simulink model "BEV"  (R2019b)
settings: Solver=ode4  StartTime=0.0  StopTime=TimeUS06  FixedStep=.1  RelTol=1e-3  EnableMultiTasking=on
PostLoadFcn:
  | addpath('ImagesBEV')
  | 
  | BEVDir = pwd;
  | 
  | cd ..\;
  | SimulinkDir = pwd;
  | addpath(SimulinkDir);
  | 
  | cd(BEVDir);
StopFcn:
  | MotorNetTorque = results.Motor.MotorNetTorque_Nm_;
  | SOC = results.Battery.SOC___;
  | BatteryPowerAtTerminals = results.Battery.BatteryPowerAtTerminals_W_;
  | VehicleSpeed = results.Glider.Velocity_mph_;
  | 
  | figure
  | scatter(VehicleSpeed.get.Data(:),MotorNetTorque.get.Data(:),'.')
  | grid on
  | box on
  | title('Motor Torque vs. Vehicle Speed')
  | xlabel('Vehicle Speed, V (mph)')
  | ylabel('Motor Torque, Tm (Nm)')
  | 
  | figure
  | scatter(VehicleSpeed.get.Data(:),BatteryPowerAtTerminals.get.Data(:))
  | grid on
  | box on
  | title('Battery Power vs. Vehicle Speed')
  | xlabel('Vehicle Speed, (mph)')
  | ylabel('Power, (kW)')
  | 
  | figure
  | plot(SOC.get.Time(:),SOC.get.Data(:))
  | grid on
  | box on
  | title('SOC vs. Time')
  | xlabel('Time (s)')
  | ylabel('SOC (%)')
  | 
  | clear MotorNetTorque SOC BatteryPowerAtTerminals VehicleSpeed ;
model workspace (MAT data in the model file):
  AccessoryLoad = 600
  C_ref = 600
  DrCycles.C505 = [0 1 2 3 4 5 6 7 8 9 10 11 ... (1012 elements, 506x2)]
  DrCycles.FTP = [0 1 2 3 4 5 6 7 8 9 10 11 ... (4956 elements, 2478x2)]
  DrCycles.UDDS = [0 1 2 3 4 5 6 7 8 9 10 11 ... (2746 elements, 1373x2)]
  DrCycles.HWFET = [0 1 2 3 4 5 6 7 8 9 10 11 ... (1532 elements, 766x2)]
  DrCycles.US06 = [0 1 2 3 4 5 6 7 8 9 10 11 ... (1194 elements, 597x2)]
  DrCycles.US06City = [0 1 2 3 4 5 6 7 8 9 10 11 ... (466 elements, 233x2)]
  DrCycles.US06Hwy = [0 1 2 3 4 5 6 7 8 9 10 11 ... (742 elements, 371x2)]
  K = 1.04716227018
  Kc_ref = 0.12
  Ki_ref = 0.01
  Kw_ref = 1.2e-05
  MDL.MotorModel.kc = 0.0452374100719
  MDL.MotorModel.ki = 0.0166666666667
  MDL.MotorModel.kw = 5.06640055941e-05
  MDL.MotorModel.C = 628.29736211
  MDL.MotorModel.MaxTrqOut = 500
  MDL.MotorModel.MaxPwrOut = 100000
  MDL.DrivelineModel.C0 = 600
  MDL.DrivelineModel.C1 = 0.012
  MDL.DrivelineModel.C2 = 4.9e-07
  MDL.DrivelineModel.G = 3.55
  MDL.DrivelineModel.Spinloss = 6
  MDL.DrivelineModel.Ftr_max = 5000
  MDL.DriverModel.Kp = 350
  MDL.DriverModel.Ki = 0
  MDL.DriverModel.Kd = 0
  MDL.DriverModel.BrakeGain = 100
  MDL.DriverModel.Ftr_Max = 5000
  MDL.DriverModel.Ptr_Max = 100000
  MDL.BrakeSys.MaxBrakeForce = 10000
  MDL.BrakeSys.RegenFraction = 0.55
  T_max = 500
  T_ref = 300
  TimeHWFET = 765
  TimeUDDS = 1372
  TimeUS06 = 596
  aeroDragCoeff = 0.38
  airDensity = 1.23
  energyCapacity = 12.6
  frontArea = 2.1
  gravity = 9.81
  inclinationAngle = 0
  inertialMassVeh = 2392
  initialSOC = 0.95
  internalResistance = 0.1
  massVeh = 2300
  openCircuitVoltage = 340
  rollingResistCoeff = 0.01
  w_max = 524
  w_ref = 834
  wheelRadius = 0.34
libraries: simulink x5, Driver_Glider_Library x2
CloseFcn:
  | rmpath(SimulinkDir);
  | rmpath('ImagesBEV')
  | clear BEVDir SimulinkDir;
settings Model: Creator=David  LastModifiedBy=valakshe
settings DataIOCC: ExternalInput=DrCycles.US06  LoadExternalInput=on  SaveFormat=Array  ReturnWorkspaceOutputs=off
settings OptimizationCC: ExpressionDepthLimit=2147483647  LifeSpan=inf
settings DebuggingCC: UnderspecifiedInitializationDetection=Classic  MergeDetectMultiDrivingBlocksExec=none  SolverPrmCheckMsg=warning  FcnCallInpInsideContextMsg=warning  StateNameClashWarn=warning  SFUnexpectedBacktrackingDiag=warning  SFNoUnconditionalDefaultTransitionDiag=warning  SFExecutionAtInitializationDiag=none  ArithmeticOperatorsInVariantConditions=warning
settings HardwareCC: ProdBitPerPointer=32  ProdBitPerSizeT=32  ProdBitPerPtrDiffT=32  ProdLargestAtomicFloat=None  ProdIntDivRoundTo=Undefined  ProdEndianess=Unspecified  ProdWordSize=32  ProdHWDeviceType=32-bit Generic
settings ModelReferenceCC: PropagateSignalLabelsOutOfModel=off
settings SFSimCC: SimUseLocalCustomCode=off  CustomCodeUndefinedFunction=UseInterfaceOnly
settings RTWCC: RTWUseLocalCustomCode=off
settings CodeAppCC: StateflowObjectComments=on
settings GRTTargetCC: TargetLangStandard=C89/C90 (ANSI)  GeneratePreprocessorConditionals=Disable all  CombineOutputUpdateFcns=off  GRTInterface=on
settings ConfigComp: CovMetricSettings=dw  CovHtmlReporting=on  CovSaveCumulativeToWorkspaceVar=on  CovSaveSingleToWorkspaceVar=on  CovExternalEMLEnable=off  CovSFcnEnable=off

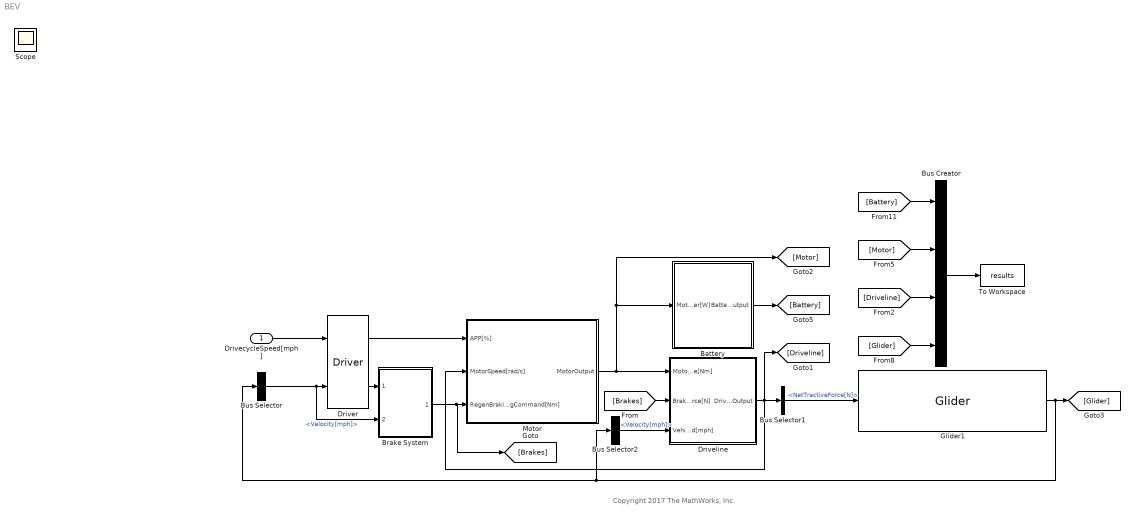
== system BEV ==
  note: Copyright 2017 The MathWorks, Inc.
  DrivecycleSpeed[mph] : Inport
  Battery : Subsystem
      mask Display: image('battery.jpg');
  Brake System : Subsystem
      mask Display: image('brakes.jpg');
  Bus Creator : BusCreator  Inputs=4
  Bus Selector : BusSelector  OutputSignals=Velocity[mph]
  Bus Selector1 : BusSelector  OutputSignals=NetTractiveForce[N]
  Bus Selector2 : BusSelector  OutputSignals=Velocity[mph]
  Driveline : Subsystem
      mask Display: image('driveline.jpg');
  Driver : Driver_Glider_Library/Driver  SystemSampleTime=-1  Latency=0  AutoFrameSizeCalculation=off
  Glider1 : Driver_Glider_Library/Glider  SystemSampleTime=-1  Latency=0  AutoFrameSizeCalculation=off
  Motor : Subsystem
      mask Display: image('motor.jpg');
  To Workspace : ToWorkspace  VariableName=results  SaveFormat=Timeseries  SampleTime=-1
  Scope : Scope
  wires:
  DrivecycleSpeed[mph]/1 -> Driver/1
  Driver/1 -> Motor/1(APP[%])
  Bus Creator/1 -> To Workspace/1
  Driver/2 -> Brake System/1(BPP[%])
  [Brakes] -> Driveline/2(BrakeForce[N])
  Brake System/1(BrakeOutput) -> [Brakes], Motor/3(RegenBrakingCommand[Nm])
  [Driveline] -> Bus Creator/3
  Driveline/1(DrivelineOutput) -> Bus Selector1/1, Motor/2(MotorSpeed[rad/s]), [Driveline]
  [Motor] -> Bus Creator/2
  Motor/1(MotorOutput) -> [Motor], Battery/1(MotorPower[W]), Driveline/1(MotorTorque[Nm])
  [Glider] -> Bus Creator/4
  Glider1/1 -> [Glider], Bus Selector/1, Bus Selector2/1
  Bus Selector/1 -> Brake System/2(VehicleSpeed[mph]), Driver/2  "<Velocity[mph]>"
  Bus Selector2/1 -> Driveline/3(VehicleSpeed[mph])  "<Velocity[mph]>"
  [Battery] -> Bus Creator/1
  Battery/1(BatteryOutput) -> [Battery]
  Bus Selector1/1 -> Glider1/1  "<NetTractiveForce[N]>"

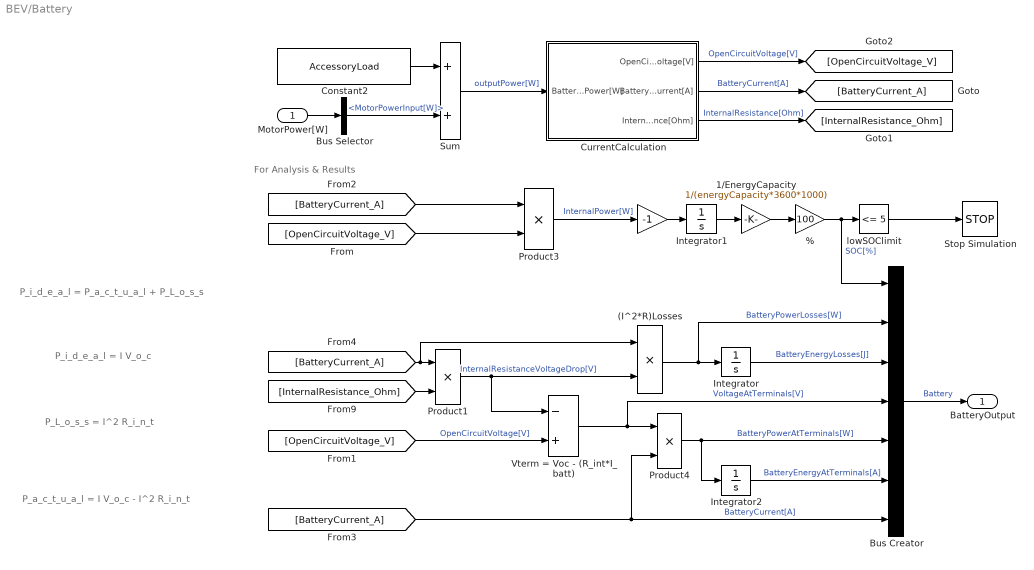
== system BEV/Battery ==
  note: For Analysis & Results
  note: P_i_d_e_a_l = I V_o_c
  note: P_i_d_e_a_l = P_a_c_t_u_a_l + P_L_o_s_s
  note: P_L_o_s_s = I^2 R_i_n_t
  note: P_a_c_t_u_a_l = I V_o_c - I^2 R_i_n_t
  MotorPower[W] : Inport
  " " : Gain  Gain=-1
  % : Gain  Gain=100
  (I^2*R)Losses : Product  RndMeth=Zero
  1/EnergyCapacity : Gain  Gain=1/(energyCapacity*3600*1000)
  Bus Creator : BusCreator  Inputs=7
  Bus Selector : BusSelector  OutputSignals=MotorPowerInput[W]
  Constant2 : Constant  Value=AccessoryLoad
  CurrentCalculation : Subsystem
  Integrator : Integrator  ZeroCross=off
  Integrator1 : Integrator  InitialCondition=energyCapacity*3600*1000*initialSOC  ZeroCross=off
  Integrator2 : Integrator
  Product1 : Product  RndMeth=Zero
  Product3 : Product  RndMeth=Zero
  Product4 : Product  RndMeth=Zero
  Stop Simulation : Stop
  Sum : Sum
  Vterm = Voc - (R_int*I_batt) : Sum  Inputs=-+
  lowSOClimit : simulink/Logic and Bit Operations/Compare To Constant  relop=<=  const=5  OutDataTypeStr=boolean
  BatteryOutput : Outport  VectorParamsAs1DForOutWhenUnconnected=off
  wires:
  Product1/1 -> (I^2*R)Losses/2, Vterm = Voc - (R_int*I_batt)/1  "InternalResistanceVoltageDrop[V]"
  (I^2*R)Losses/1 -> Bus Creator/2, Integrator/1  "BatteryPowerLosses[W]"
  Integrator/1 -> Bus Creator/3  "BatteryEnergyLosses[J]"
  Product3/1 -> " "/1  "InternalPower[W]"
  Integrator1/1 -> 1/EnergyCapacity/1
  Constant2/1 -> Sum/1
  Bus Creator/1 -> BatteryOutput/1  "Battery"
  1/EnergyCapacity/1 -> %/1
  MotorPower[W]/1 -> Bus Selector/1
  Sum/1 -> CurrentCalculation/1(BatteryPower[W])  "outputPower[W]"
  " "/1 -> Integrator1/1
  Bus Selector/1 -> Sum/2  "<MotorPowerInput[W]>"
  [OpenCircuitVoltage_V] -> Product3/2
  CurrentCalculation/1(OpenCircuitVoltage[V]) -> [OpenCircuitVoltage_V]  "OpenCircuitVoltage[V]"
  [OpenCircuitVoltage_V] -> Vterm = Voc - (R_int*I_batt)/2  "OpenCircuitVoltage[V]"
  [BatteryCurrent_A] -> Product3/1
  [BatteryCurrent_A] -> Bus Creator/7, Product4/2  "BatteryCurrent[A]"
  [BatteryCurrent_A] -> (I^2*R)Losses/1, Product1/1
  Vterm = Voc - (R_int*I_batt)/1 -> Bus Creator/4, Product4/1  "VoltageAtTerminals[V]"
  CurrentCalculation/2(BatteryCurrent[A]) -> [BatteryCurrent_A]  "BatteryCurrent[A]"
  CurrentCalculation/3(InternalResistance[Ohm]) -> [InternalResistance_Ohm]  "InternalResistance[Ohm]"
  [InternalResistance_Ohm] -> Product1/2
  Product4/1 -> Bus Creator/5, Integrator2/1  "BatteryPowerAtTerminals[W]"
  Integrator2/1 -> Bus Creator/6  "BatteryEnergyAtTerminals[A]"
  %/1 -> lowSOClimit/1, Bus Creator/1  "SOC[%]"
  lowSOClimit/1 -> Stop Simulation/1

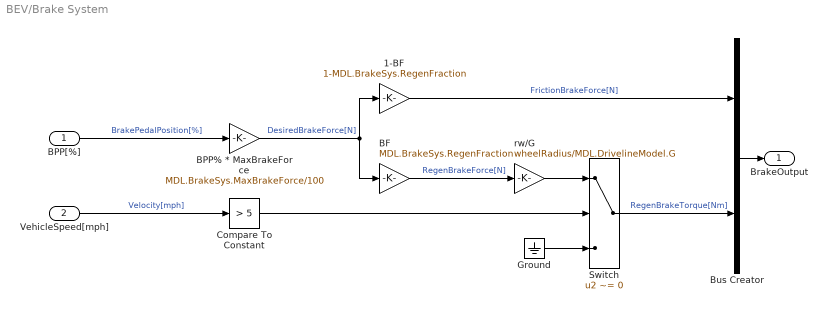
== system BEV/Brake System ==
  BPP[%] : Inport
  VehicleSpeed[mph] : Inport  Port=2
  1-BF : Gain  Gain=1-MDL.BrakeSys.RegenFraction
  BF : Gain  Gain=MDL.BrakeSys.RegenFraction
  BPP% * MaxBrakeForce : Gain  Gain=MDL.BrakeSys.MaxBrakeForce/100
  Bus Creator : BusCreator  Inputs=2
  Compare To Constant : simulink/Logic and Bit Operations/Compare To Constant  relop=>  const=5  OutDataTypeStr=boolean
  Ground : Ground
  Switch : Switch  Criteria=u2 ~= 0
  rw/G : Gain  Gain=wheelRadius/MDL.DrivelineModel.G
  BrakeOutput : Outport  VectorParamsAs1DForOutWhenUnconnected=off
  wires:
  Bus Creator/1 -> BrakeOutput/1
  BPP[%]/1 -> BPP% * MaxBrakeForce/1  "BrakePedalPosition[%]"
  BPP% * MaxBrakeForce/1 -> BF/1, 1-BF/1  "DesiredBrakeForce[N]"
  BF/1 -> rw/G/1  "RegenBrakeForce[N]"
  1-BF/1 -> Bus Creator/1  "FrictionBrakeForce[N]"
  rw/G/1 -> Switch/1
  VehicleSpeed[mph]/1 -> Compare To Constant/1  "Velocity[mph]"
  Ground/1 -> Switch/3
  Switch/1 -> Bus Creator/2  "RegenBrakeTorque[Nm]"
  Compare To Constant/1 -> Switch/2

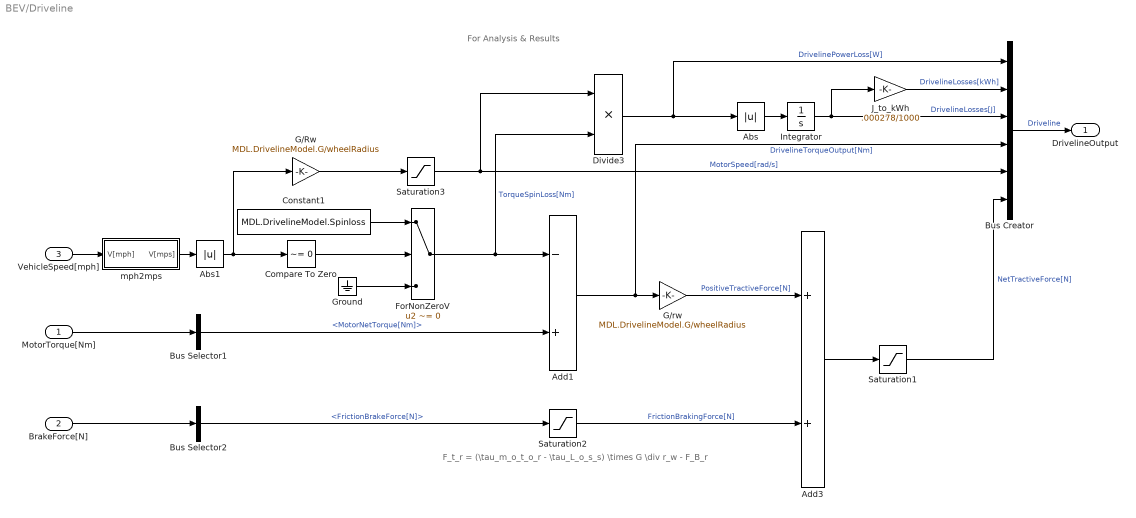
== system BEV/Driveline ==
  note: For Analysis & Results
  note: F_t_r = (\tau_m_o_t_o_r - \tau_L_o_s_s) \times G \div r_w - F_B_r
  MotorTorque[Nm] : Inport
  BrakeForce[N] : Inport  Port=2
  VehicleSpeed[mph] : Inport  Port=3
  Abs : Abs  ZeroCross=off
  Abs1 : Abs  ZeroCross=off
  Add1 : Sum  Inputs=-+
  Add3 : Sum
  Bus Creator : BusCreator  Inputs=6
  Bus Selector1 : BusSelector  OutputSignals=MotorNetTorque[Nm]
  Bus Selector2 : BusSelector  OutputSignals=FrictionBrakeForce[N]
  Compare To Zero : simulink/Logic and Bit Operations/Compare To Zero  relop=~=  OutDataTypeStr=boolean
  Constant1 : Constant  Value=MDL.DrivelineModel.Spinloss
  Divide3 : Product  Inputs=**
  ForNonZeroV : Switch  Criteria=u2 ~= 0  ZeroCross=off
  G/Rw : Gain  Gain=MDL.DrivelineModel.G/wheelRadius
  G/rw : Gain  Gain=MDL.DrivelineModel.G/wheelRadius
  Ground : Ground
  Integrator : Integrator  ZeroCross=off
  J_to_kWh : Gain  Gain=.000278/1000
  Saturation1 : Saturate  UpperLimit=5000  LowerLimit=-10000  ZeroCross=off
  Saturation2 : Saturate  UpperLimit=0  LowerLimit=-10000  ZeroCross=off
  Saturation3 : Saturate  UpperLimit=inf  LowerLimit=0.00001  ZeroCross=off
  mph2mps : Subsystem
  DrivelineOutput : Outport  VectorParamsAs1DForOutWhenUnconnected=off
  wires:
  G/rw/1 -> Add3/1  "PositiveTractiveForce[N]"
  Add3/1 -> Saturation1/1
  Abs/1 -> Integrator/1
  BrakeForce[N]/1 -> Bus Selector2/1
  Saturation2/1 -> Add3/2  "FrictionBrakingForce[N]"
  MotorTorque[Nm]/1 -> Bus Selector1/1
  G/Rw/1 -> Saturation3/1
  VehicleSpeed[mph]/1 -> mph2mps/1(V[mph])
  ForNonZeroV/1 -> Divide3/2, Add1/1  "TorqueSpinLoss[Nm]"
  Add1/1 -> Bus Creator/4, G/rw/1  "DrivelineTorqueOutput[Nm]"
  Saturation3/1 -> Divide3/1, Bus Creator/5  "MotorSpeed[rad/s]"
  Divide3/1 -> Bus Creator/1, Abs/1  "DrivelinePowerLoss[W]"
  Saturation1/1 -> Bus Creator/6  "NetTractiveForce[N]"
  Abs1/1 -> Compare To Zero/1, G/Rw/1
  Bus Selector2/1 -> Saturation2/1  "<FrictionBrakeForce[N]>"
  J_to_kWh/1 -> Bus Creator/2  "DrivelineLosses[kWh]"
  Ground/1 -> ForNonZeroV/3
  Constant1/1 -> ForNonZeroV/1
  Bus Creator/1 -> DrivelineOutput/1  "Driveline"
  Integrator/1 -> J_to_kWh/1, Bus Creator/3  "DrivelineLosses[J]"
  Bus Selector1/1 -> Add1/2  "<MotorNetTorque[Nm]>"
  Compare To Zero/1 -> ForNonZeroV/2
  mph2mps/1(V[mps]) -> Abs1/1

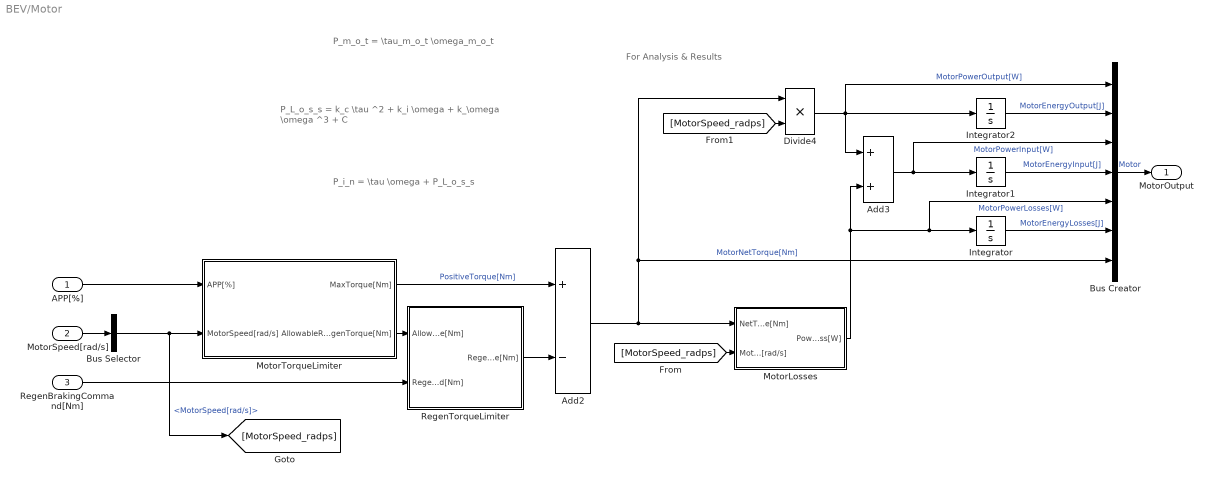
== system BEV/Motor ==
  note: P_i_n = \tau \omega + P_L_o_s_s
  note: For Analysis & Results
  note: P_L_o_s_s = k_c \tau ^2 + k_i \omega + k_\omega \omega ^3 + C
  note: P_m_o_t = \tau_m_o_t \omega_m_o_t
  APP[%] : Inport
  MotorSpeed[rad/s] : Inport  Port=2
  RegenBrakingCommand[Nm] : Inport  Port=3
  Add2 : Sum  Inputs=+-
  Add3 : Sum
  Bus Creator : BusCreator  Inputs=7
  Bus Selector : BusSelector  OutputSignals=MotorSpeed[rad/s]
  Divide4 : Product  Inputs=**
  Integrator : Integrator  ZeroCross=off
  Integrator1 : Integrator  ZeroCross=off
  Integrator2 : Integrator  ZeroCross=off
  MotorLosses : Subsystem
  MotorTorqueLimiter : Subsystem
  RegenTorqueLimiter : Subsystem
  MotorOutput : Outport  VectorParamsAs1DForOutWhenUnconnected=off
  wires:
  Add3/1 -> Bus Creator/3, Integrator1/1  "MotorPowerInput[W]"
  Divide4/1 -> Bus Creator/1, Add3/1, Integrator2/1  "MotorPowerOutput[W]"
  [MotorSpeed_radps] -> Divide4/2
  Integrator1/1 -> Bus Creator/4  "MotorEnergyInput[J]"
  Integrator2/1 -> Bus Creator/2  "MotorEnergyOutput[J]"
  Add2/1 -> MotorLosses/1(NetTorque[Nm]), Divide4/1, Bus Creator/7  "MotorNetTorque[Nm]"
  MotorTorqueLimiter/1(MaxTorque[Nm]) -> Add2/1  "PositiveTorque[Nm]"
  APP[%]/1 -> MotorTorqueLimiter/1(APP[%])
  MotorLosses/1(PowerLoss[W]) -> Bus Creator/5, Integrator/1, Add3/2  "MotorPowerLosses[W]"
  RegenBrakingCommand[Nm]/1 -> RegenTorqueLimiter/2(RegenBrakeCommand[Nm])
  MotorTorqueLimiter/2(AllowableRegenTorque[Nm]) -> RegenTorqueLimiter/1(AllowableRegenTorque[Nm])
  RegenTorqueLimiter/1(RegenTorque[Nm]) -> Add2/2
  [MotorSpeed_radps] -> MotorLosses/2(MotorSpeed[rad/s])
  Bus Creator/1 -> MotorOutput/1  "Motor"
  Integrator/1 -> Bus Creator/6  "MotorEnergyLosses[J]"
  MotorSpeed[rad/s]/1 -> Bus Selector/1
  Bus Selector/1 -> MotorTorqueLimiter/2(MotorSpeed[rad/s]), [MotorSpeed_radps]  "<MotorSpeed[rad/s]>"

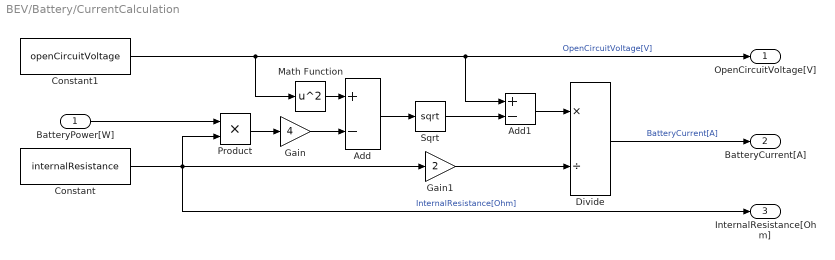
== system BEV/Battery/CurrentCalculation ==
  BatteryPower[W] : Inport
  Add : Sum  Inputs=+-
  Add1 : Sum  Inputs=+-
  Constant : Constant  Value=internalResistance
  Constant1 : Constant  Value=openCircuitVoltage
  Divide : Product  Inputs=*/
  Gain : Gain  Gain=4
  Gain1 : Gain  Gain=2
  Math Function : Math  Operator=square  SaturateOnIntegerOverflow=on
  Product : Product  RndMeth=Zero
  Sqrt : Sqrt  SaturateOnIntegerOverflow=on
  OpenCircuitVoltage[V] : Outport  VectorParamsAs1DForOutWhenUnconnected=off
  BatteryCurrent[A] : Outport  Port=2  VectorParamsAs1DForOutWhenUnconnected=off
  InternalResistance[Ohm] : Outport  Port=3  VectorParamsAs1DForOutWhenUnconnected=off
  wires:
  BatteryPower[W]/1 -> Product/1
  Constant/1 -> InternalResistance[Ohm]/1, Gain1/1, Product/2  "InternalResistance[Ohm]"
  Product/1 -> Gain/1
  Constant1/1 -> Math Function/1, OpenCircuitVoltage[V]/1, Add1/1  "OpenCircuitVoltage[V]"
  Math Function/1 -> Add/1
  Gain/1 -> Add/2
  Sqrt/1 -> Add1/2
  Add/1 -> Sqrt/1
  Add1/1 -> Divide/1
  Gain1/1 -> Divide/2
  Divide/1 -> BatteryCurrent[A]/1  "BatteryCurrent[A]"

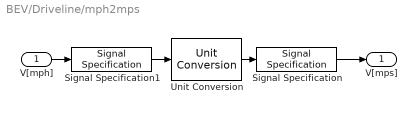
== system BEV/Driveline/mph2mps ==
  V[mph] : Inport
  Signal Specification : SignalSpecification  Unit=m/s
  Signal Specification1 : SignalSpecification  Unit=mile/hr
  Unit Conversion : UnitConversion
  V[mps] : Outport  VectorParamsAs1DForOutWhenUnconnected=off
  wires:
  V[mph]/1 -> Signal Specification1/1
  Unit Conversion/1 -> Signal Specification/1
  Signal Specification1/1 -> Unit Conversion/1
  Signal Specification/1 -> V[mps]/1

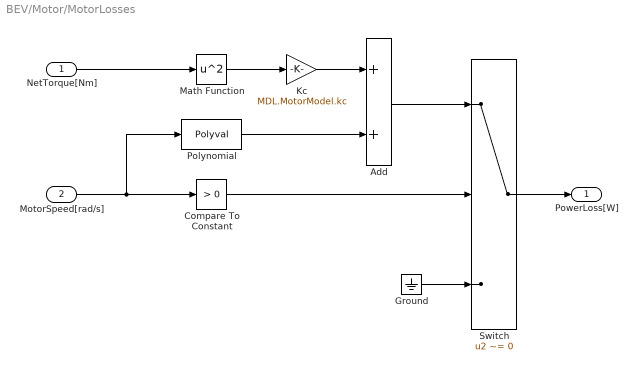
== system BEV/Motor/MotorLosses ==
  NetTorque[Nm] : Inport
  MotorSpeed[rad/s] : Inport  Port=2
  Add : Sum
  Compare To Constant : simulink/Logic and Bit Operations/Compare To Constant  relop=>  const=0  OutDataTypeStr=boolean
  Ground : Ground
  Kc : Gain  Gain=MDL.MotorModel.kc
  Math Function : Math  Operator=square  SaturateOnIntegerOverflow=on
  Polynomial : Polyval  Coefs=[MDL.MotorModel.kw , 0 ,MDL.MotorModel.ki, MDL.MotorModel.C]
  Switch : Switch  Criteria=u2 ~= 0  ZeroCross=off
  PowerLoss[W] : Outport  VectorParamsAs1DForOutWhenUnconnected=off
  wires:
  NetTorque[Nm]/1 -> Math Function/1
  Math Function/1 -> Kc/1
  Kc/1 -> Add/1
  MotorSpeed[rad/s]/1 -> Polynomial/1, Compare To Constant/1
  Ground/1 -> Switch/3
  Switch/1 -> PowerLoss[W]/1
  Polynomial/1 -> Add/2
  Add/1 -> Switch/1
  Compare To Constant/1 -> Switch/2

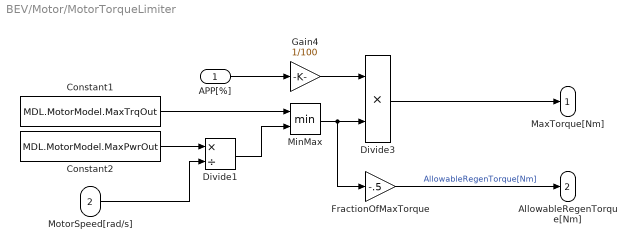
== system BEV/Motor/MotorTorqueLimiter ==
  APP[%] : Inport
  MotorSpeed[rad/s] : Inport  Port=2
  Constant1 : Constant  Value=MDL.MotorModel.MaxTrqOut
  Constant2 : Constant  Value=MDL.MotorModel.MaxPwrOut
  Divide1 : Product  Inputs=*/
  Divide3 : Product  Inputs=**
  FractionOfMaxTorque : Gain  Gain=-.5
  Gain4 : Gain  Gain=1/100
  MinMax : MinMax  Inputs=2
  MaxTorque[Nm] : Outport  VectorParamsAs1DForOutWhenUnconnected=off
  AllowableRegenTorque[Nm] : Outport  Port=2  VectorParamsAs1DForOutWhenUnconnected=off
  wires:
  Constant1/1 -> MinMax/1
  MinMax/1 -> FractionOfMaxTorque/1, Divide3/2
  Gain4/1 -> Divide3/1
  APP[%]/1 -> Gain4/1
  Divide3/1 -> MaxTorque[Nm]/1
  Constant2/1 -> Divide1/1
  Divide1/1 -> MinMax/2
  MotorSpeed[rad/s]/1 -> Divide1/2
  FractionOfMaxTorque/1 -> AllowableRegenTorque[Nm]/1  "AllowableRegenTorque[Nm]"

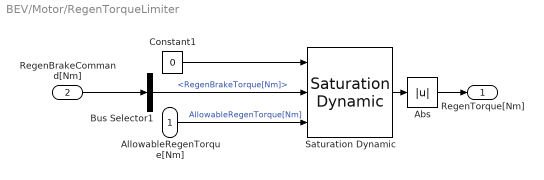
== system BEV/Motor/RegenTorqueLimiter ==
  AllowableRegenTorque[Nm] : Inport
  RegenBrakeCommand[Nm] : Inport  Port=2
  Abs : Abs
  Bus Selector1 : BusSelector  OutputSignals=RegenBrakeTorque[Nm]
  Constant1 : Constant  Value=0
  Saturation Dynamic : simulink/Discontinuities/Saturation Dynamic  OutMin=[]  OutMax=[]  OutDataTypeStr=Inherit: Same as second input  OutDataType=fixdt(1, 16)  OutScaling=2^-10  DoSatur=off
  RegenTorque[Nm] : Outport  VectorParamsAs1DForOutWhenUnconnected=off
  wires:
  AllowableRegenTorque[Nm]/1 -> Saturation Dynamic/3  "AllowableRegenTorque[Nm]"
  Constant1/1 -> Saturation Dynamic/1
  Bus Selector1/1 -> Saturation Dynamic/2  "<RegenBrakeTorque[Nm]>"
  RegenBrakeCommand[Nm]/1 -> Bus Selector1/1
  Saturation Dynamic/1 -> Abs/1
  Abs/1 -> RegenTorque[Nm]/1
